simulink model "Hito1"  (R2022b)
settings: Solver=FixedStepAuto  StartTime=0.0  StopTime=inf  RelTol=1e-3  EnableMultiTasking=on
libraries: simulink x8
settings Model: ExtModeTrigDuration=2  Creator=miriamfreiriasanjuan  LastModifiedBy=miriamfreiriasanjuan
settings SolverCC: AutoInsertRateTranBlk=on
settings OptimizationCC: EnhancedBackFolding=on  PassReuseOutputArgsAs=Individual arguments  ZeroExternalMemoryAtStartup=off  ZeroInternalMemoryAtStartup=off  MaxStackSize=64  OptimizeBlockOrder=speed  DifferentSizesBufferReuse=on  OptimizationCustomize=off  EfficientTunableParamExpr=on
settings DebuggingCC: ParameterOverflowMsg=none  ParameterPrecisionLossMsg=none  ParameterTunabilityLossMsg=error
settings HardwareCC: ProdBitPerInt=16  ProdBitPerPointer=16  ProdBitPerSizeT=16  ProdBitPerPtrDiffT=16  ProdLargestAtomicFloat=None  ProdWordSize=8  ProdHWDeviceType=Atmel->AVR
settings SFSimCC: MATLABDynamicMemAlloc=off
settings RTWCC: Description=Embedded Coder  SystemTargetFile=ert.tlc  HardwareBoard=Arduino Mega 2560  TLCOptions=-aInlineSetEventsForThisBaseRateFcn=TLC_FALSE -aSuppressMultiTaskScheduler=TLC_FALSE -aRateBasedStepFcn=1  TemplateMakefile=ert_default_tmf  Toolchain=Arduino AVR  BuildConfiguration=Faster Runs
settings CodeAppCC: ForceParamTrailComments=on  IgnoreCustomStorageClasses=off  OperatorAnnotations=on  SimulinkDataObjDesc=on  SFDataObjDesc=on  InsertBlockDesc=on
settings ERTTargetCC: SupportContinuousTime=on  SupportVariableSizeSignals=on  ExtModeTransport=3  ExtModeStaticAlloc=on  ExtModeAutomaticAllocSize=off  ExtModeStaticAllocSize=2048  ExtModeMexFile=ext_xcp  ExtModeIntrfLevel=Level2 - Open

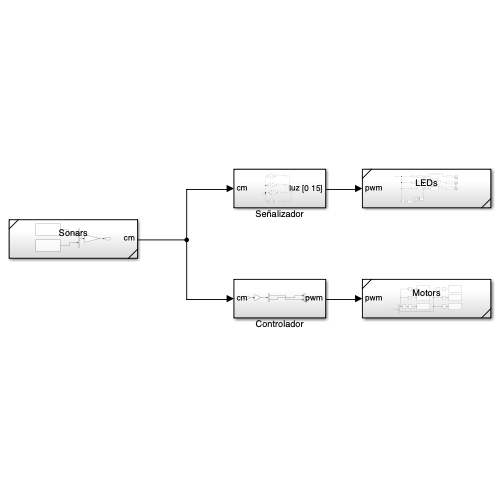
[thumbnail: Simulink's stored preview of the top-level diagram]
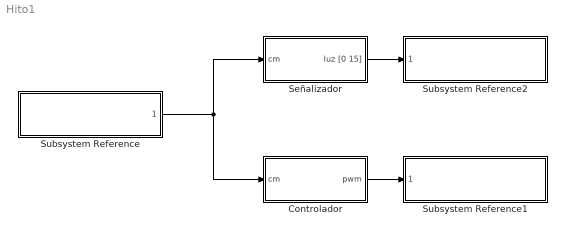
== system Hito1 ==
  Controlador : Subsystem
      settings: LibrarySourceBlock=|
      | hdlsllib/Ports &
      | Subsystems/Subsystem
  Señalizador : Subsystem
      settings: LibrarySourceBlock=|
      | hdlsllib/Ports &
      | Subsystems/Subsystem
  Subsystem Reference : Subsystem  ReferencedSubsystem=Sonars
  Subsystem Reference1 : Subsystem  ReferencedSubsystem=Motors
  Subsystem Reference2 : Subsystem  ReferencedSubsystem=LEDs
  wires:
  Subsystem Reference/1 -> Controlador/1(cm), Señalizador/1(cm)
  Señalizador/1(luz [0 15]) -> Subsystem Reference2/1
  Controlador/1(pwm) -> Subsystem Reference1/1

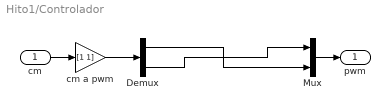
== system Hito1/Controlador ==
  cm : Inport
  Demux : Demux  Outputs=2
  Mux : Mux  Inputs=2
  cm a pwm : Gain  Gain=[1 1]  ParamDataTypeStr=int16
  pwm : Outport
  wires:
  Mux/1 -> pwm/1
  cm/1 -> cm a pwm/1
  Demux/1 -> Mux/2
  Demux/2 -> Mux/1
  cm a pwm/1 -> Demux/1

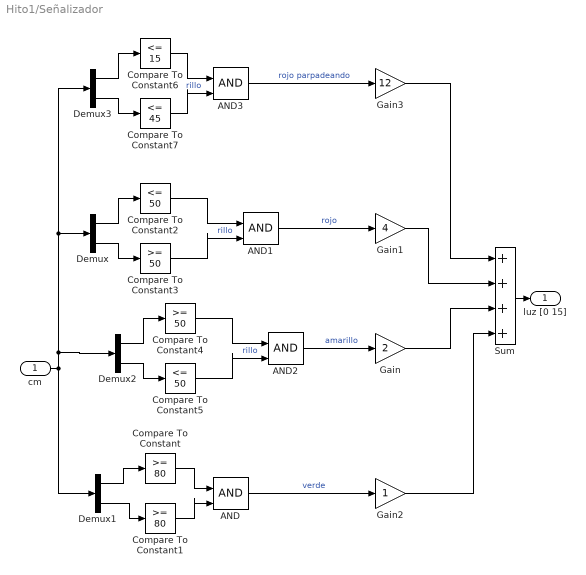
== system Hito1/Señalizador ==
  cm : Inport
  AND{,1..3} (4 alike) : Logic  IconShape=distinctive  AllPortsSameDT=off  OutDataTypeStr=boolean
  Compare To Constant : simulink/Logic and Bit Operations/Compare To Constant  relop=>=  const=80  OutDataTypeStr=boolean
  Compare To Constant1 : simulink/Logic and Bit Operations/Compare To Constant  relop=>=  const=80  OutDataTypeStr=boolean
  Compare To Constant2 : simulink/Logic and Bit Operations/Compare To Constant  relop=<=  const=50  OutDataTypeStr=boolean
  Compare To Constant3 : simulink/Logic and Bit Operations/Compare To Constant  relop=>=  const=50  OutDataTypeStr=boolean
  Compare To Constant4 : simulink/Logic and Bit Operations/Compare To Constant  relop=>=  const=50  OutDataTypeStr=boolean
  Compare To Constant5 : simulink/Logic and Bit Operations/Compare To Constant  relop=<=  const=50  OutDataTypeStr=boolean
  Compare To Constant6 : simulink/Logic and Bit Operations/Compare To Constant  relop=<=  const=15  OutDataTypeStr=boolean
  Compare To Constant7 : simulink/Logic and Bit Operations/Compare To Constant  relop=<=  const=45  OutDataTypeStr=boolean
  Demux{,1..3} (4 alike) : Demux  Outputs=2
  Gain : Gain  Gain=2
  Gain1 : Gain  Gain=4
  Gain2 : Gain
  Gain3 : Gain  Gain=12
  Sum : Sum  Inputs=++++
  luz [0 15] : Outport
  wires:
  Demux1/1 -> Compare To Constant/1
  Demux1/2 -> Compare To Constant1/1
  Compare To Constant/1 -> AND/1
  Compare To Constant1/1 -> AND/2
  Demux/1 -> Compare To Constant2/1
  Demux/2 -> Compare To Constant3/1
  Compare To Constant2/1 -> AND1/1
  Compare To Constant3/1 -> AND1/2  "rillo"
  AND1/1 -> Gain1/1  "rojo"
  Compare To Constant5/1 -> AND2/2  "rillo"
  Demux2/2 -> Compare To Constant5/1
  Demux2/1 -> Compare To Constant4/1
  Compare To Constant4/1 -> AND2/1
  AND2/1 -> Gain/1  "amarillo"
  cm/1 -> Demux1/1, Demux2/1, Demux3/1, Demux/1
  Compare To Constant7/1 -> AND3/2  "rillo"
  Demux3/2 -> Compare To Constant7/1
  Demux3/1 -> Compare To Constant6/1
  Compare To Constant6/1 -> AND3/1
  AND3/1 -> Gain3/1  "rojo parpadeando"
  AND/1 -> Gain2/1  "verde"
  Sum/1 -> luz [0 15]/1
  Gain3/1 -> Sum/1
  Gain1/1 -> Sum/2
  Gain/1 -> Sum/3
  Gain2/1 -> Sum/4
